simulink model "Inverter_32V_2A"  (R2025b)
settings: Solver=VariableStepAuto  StartTime=0.0  StopTime=0.3  FixedStep=SPWM_Ts  RelTol=1e-3
model workspace (MAT data in the model file):
  AC_LoadResistance = 9.23760430703
  AD_TimeConstant = 0.00025
  AD_a = [1 -0.881765205117]
  AD_b = [2.95586987209 -2.95586987209]
  CL_AAComp = 1.00249999972
  CL_Kaw = 20
  CL_Ki = 1.6
  CL_Kp = 0.005
  CL_N = 200
  CL_Ts = 0.0001
  CL_Vref = 32
  CL_faa = 1000
  CL_fp = 50
  CL_mff = 0.94
  CL_mmax = 1
  CommonModeBias = 0.15
  CommonModeKp = 0.02
  CommonModeShift = 1
  ControlStartTime = 0.06
  DampingCapuF = 4.7
  DampingResistance = 30
  DeadtimeComp = 0.08
  DeadtimeCurrentBand = 0.2
  DutyFeedforward = 0
  DutyMax = 0.75
  FilterDCR = 0.3
  KiCurrentLoop = 5
  KiVoltageLoop = 5
  KpCurrentLoop = 0.08
  KpVoltageLoop = 0.2
  LoadConnectTime = 0.18
  MainFilterCapuF = 4.7
  PR_Gain = 1.25
  PR_a10 = [1 -1.99838562653 0.999372033695]
  PR_a11 = [1 -1.99817857535 0.999372066214]
  PR_a13 = [1 -1.99770539603 0.999372140529]
  PR_a16 = [1 -1.99684804391 0.99937227518]
  PR_a17 = [1 -1.99652293757 0.99937232624]
  PR_a19 = [1 -1.9958137982 0.999372437614]
  PR_a2 = [1 -1.99933241937 0.999371884997]
  PR_a4 = [1 -1.99921404574 0.999371903588]
  PR_a5 = [1 -1.99912527012 0.99937191753]
  PR_a7 = [1 -1.9988885544 0.999371954708]
  PR_a8 = [1 -1.99874062131 0.999371977941]
  PR_b10 = [0.236875635534 -0.472442728614 0.23556709308]
  PR_b11 = [0.215389811794 -0.429471148895 0.214081337101]
  PR_b13 = [0.182331988259 -0.363355656682 0.181023668423]
  PR_b16 = [0.148235597863 -0.295163156474 0.146927558611]
  PR_b17 = [0.139542977111 -0.277778021366 0.138235044255]
  PR_b19 = [0.124900915012 -0.248494129248 0.123593214235]
  PR_b2 = [0.425928775502 -0.847596177142 0.42166740164]
  PR_b4 = [0.279572378961 -0.55553023994 0.275957860979]
  PR_b5 = [0.246657018631 -0.490084248228 0.243427229597]
  PR_b7 = [0.202908225742 -0.403457656245 0.200549430503]
  PR_b8 = [0.186290317354 -0.370698545076 0.184408227722]
  PrechargeBypassTime = 0.16
  PrechargeResistance = 47
  RegenerativeMode = 1
  ReturnCurrent = 2
  ReturnRampTime = 0.08
  ReturnTs = 1e-05
  SPWM_Ndead = 10
  SPWM_Tdead = 2e-06
  SPWM_Ts = 2e-07
  SPWM_Vgate = 10
  SPWM_f1 = 50
  SPWM_fs = 20000
  SPWM_m = 0.8
  VoltageRampRate = 100
  op_snapshot1 : opcond.OperatingPoint (value not decoded)
  testadd = 0
undefined symbols (not defined in the file): DiscIntNeverNeededParam, dspblkCoreblockFVToolHelper, gcbh
libraries: fl_lib x31, ee_lib x30, nesl_utility x26, simulink x1
(part 2 of 2)

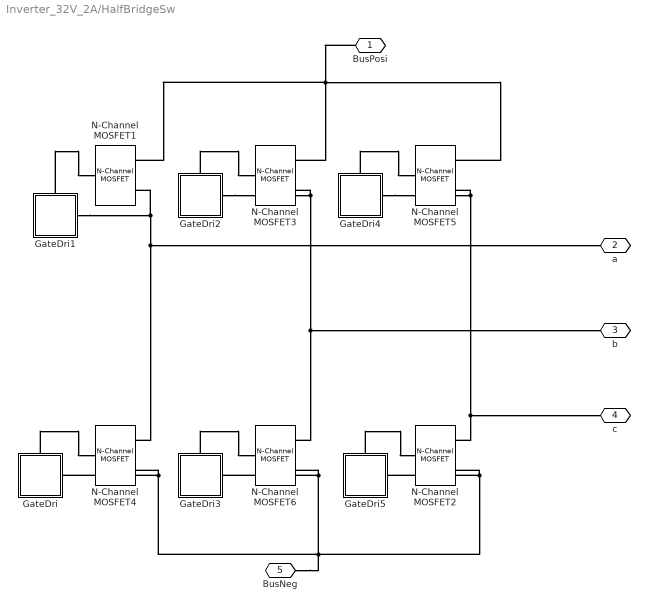
== system Inverter_32V_2A/HalfBridgeSw ==
  GateDri : Subsystem
      settings: PortSchema="{\"entries\":[{\"content\":{\"sides\":[{\"content\":{\"connectorIds\":[\"LConn1\"]},\"type\":\"ConnectorPlacement.EquallySpacedRectSide\",\"uuid\":\"5ec2b66a-2e5f-4a29-ad7d-11e5a28469f4\"},{\"content\":{\"side\":\"RIGHT\"},\"type\":\"ConnectorPlacement.EquallySpacedRectSide\",\"uuid\":\"968cf12b-ade8-46ac-9f94-1e8ea2f3f677\"},{\"content\":{\"side\":\"TOP\"},\"type\":\"ConnectorPlacement.EquallySpacedRectSide\",\"uuid\":\"41030f6a-5ac0-4230-aa4b-0c03378f97d6\"},{\"content\":{\"connectorIds\":[\"RConn1\"],\"side\":\"BOTTOM\"},\"type\":\"ConnectorPlacement.EquallySpacedRectSide\",\"uuid\":\"8f964c8e-6f21-4ad0-8f7c-edbb0b22c660\"}]},\"type\":\"ConnectorPlacement.EquallySpacedConnector\",\"uuid\":\"dccfb76b-3882-476d-8e51-da801e2932e6\"}],\"packageUris\":[\"http://schema.mathworks.com/mf0/Connector/R2020b\"],\"version\":\"1.0\"}"
  GateDri1 : Subsystem
      settings: PortSchema="{\"entries\":[{\"content\":{\"sides\":[{\"content\":{\"connectorIds\":[\"LConn1\"]},\"type\":\"ConnectorPlacement.EquallySpacedRectSide\",\"uuid\":\"5ec2b66a-2e5f-4a29-ad7d-11e5a28469f4\"},{\"content\":{\"side\":\"RIGHT\"},\"type\":\"ConnectorPlacement.EquallySpacedRectSide\",\"uuid\":\"968cf12b-ade8-46ac-9f94-1e8ea2f3f677\"},{\"content\":{\"side\":\"TOP\"},\"type\":\"ConnectorPlacement.EquallySpacedRectSide\",\"uuid\":\"41030f6a-5ac0-4230-aa4b-0c03378f97d6\"},{\"content\":{\"connectorIds\":[\"RConn1\"],\"side\":\"BOTTOM\"},\"type\":\"ConnectorPlacement.EquallySpacedRectSide\",\"uuid\":\"8f964c8e-6f21-4ad0-8f7c-edbb0b22c660\"}]},\"type\":\"ConnectorPlacement.EquallySpacedConnector\",\"uuid\":\"dccfb76b-3882-476d-8e51-da801e2932e6\"}],\"packageUris\":[\"http://schema.mathworks.com/mf0/Connector/R2020b\"],\"version\":\"1.0\"}"
  GateDri2 : Subsystem
      settings: PortSchema="{\"entries\":[{\"content\":{\"sides\":[{\"content\":{\"connectorIds\":[\"LConn1\"]},\"type\":\"ConnectorPlacement.EquallySpacedRectSide\",\"uuid\":\"5ec2b66a-2e5f-4a29-ad7d-11e5a28469f4\"},{\"content\":{\"side\":\"RIGHT\"},\"type\":\"ConnectorPlacement.EquallySpacedRectSide\",\"uuid\":\"968cf12b-ade8-46ac-9f94-1e8ea2f3f677\"},{\"content\":{\"side\":\"TOP\"},\"type\":\"ConnectorPlacement.EquallySpacedRectSide\",\"uuid\":\"41030f6a-5ac0-4230-aa4b-0c03378f97d6\"},{\"content\":{\"connectorIds\":[\"RConn1\"],\"side\":\"BOTTOM\"},\"type\":\"ConnectorPlacement.EquallySpacedRectSide\",\"uuid\":\"8f964c8e-6f21-4ad0-8f7c-edbb0b22c660\"}]},\"type\":\"ConnectorPlacement.EquallySpacedConnector\",\"uuid\":\"dccfb76b-3882-476d-8e51-da801e2932e6\"}],\"packageUris\":[\"http://schema.mathworks.com/mf0/Connector/R2020b\"],\"version\":\"1.0\"}"
  GateDri3 : Subsystem
      settings: PortSchema="{\"entries\":[{\"content\":{\"sides\":[{\"content\":{\"connectorIds\":[\"LConn1\"]},\"type\":\"ConnectorPlacement.EquallySpacedRectSide\",\"uuid\":\"5ec2b66a-2e5f-4a29-ad7d-11e5a28469f4\"},{\"content\":{\"side\":\"RIGHT\"},\"type\":\"ConnectorPlacement.EquallySpacedRectSide\",\"uuid\":\"968cf12b-ade8-46ac-9f94-1e8ea2f3f677\"},{\"content\":{\"side\":\"TOP\"},\"type\":\"ConnectorPlacement.EquallySpacedRectSide\",\"uuid\":\"41030f6a-5ac0-4230-aa4b-0c03378f97d6\"},{\"content\":{\"connectorIds\":[\"RConn1\"],\"side\":\"BOTTOM\"},\"type\":\"ConnectorPlacement.EquallySpacedRectSide\",\"uuid\":\"8f964c8e-6f21-4ad0-8f7c-edbb0b22c660\"}]},\"type\":\"ConnectorPlacement.EquallySpacedConnector\",\"uuid\":\"dccfb76b-3882-476d-8e51-da801e2932e6\"}],\"packageUris\":[\"http://schema.mathworks.com/mf0/Connector/R2020b\"],\"version\":\"1.0\"}"
  GateDri4 : Subsystem
      settings: PortSchema="{\"entries\":[{\"content\":{\"sides\":[{\"content\":{\"connectorIds\":[\"LConn1\"]},\"type\":\"ConnectorPlacement.EquallySpacedRectSide\",\"uuid\":\"5ec2b66a-2e5f-4a29-ad7d-11e5a28469f4\"},{\"content\":{\"side\":\"RIGHT\"},\"type\":\"ConnectorPlacement.EquallySpacedRectSide\",\"uuid\":\"968cf12b-ade8-46ac-9f94-1e8ea2f3f677\"},{\"content\":{\"side\":\"TOP\"},\"type\":\"ConnectorPlacement.EquallySpacedRectSide\",\"uuid\":\"41030f6a-5ac0-4230-aa4b-0c03378f97d6\"},{\"content\":{\"connectorIds\":[\"RConn1\"],\"side\":\"BOTTOM\"},\"type\":\"ConnectorPlacement.EquallySpacedRectSide\",\"uuid\":\"8f964c8e-6f21-4ad0-8f7c-edbb0b22c660\"}]},\"type\":\"ConnectorPlacement.EquallySpacedConnector\",\"uuid\":\"dccfb76b-3882-476d-8e51-da801e2932e6\"}],\"packageUris\":[\"http://schema.mathworks.com/mf0/Connector/R2020b\"],\"version\":\"1.0\"}"
  GateDri5 : Subsystem
      settings: PortSchema="{\"entries\":[{\"content\":{\"sides\":[{\"content\":{\"connectorIds\":[\"LConn1\"]},\"type\":\"ConnectorPlacement.EquallySpacedRectSide\",\"uuid\":\"5ec2b66a-2e5f-4a29-ad7d-11e5a28469f4\"},{\"content\":{\"side\":\"RIGHT\"},\"type\":\"ConnectorPlacement.EquallySpacedRectSide\",\"uuid\":\"968cf12b-ade8-46ac-9f94-1e8ea2f3f677\"},{\"content\":{\"side\":\"TOP\"},\"type\":\"ConnectorPlacement.EquallySpacedRectSide\",\"uuid\":\"41030f6a-5ac0-4230-aa4b-0c03378f97d6\"},{\"content\":{\"connectorIds\":[\"RConn1\"],\"side\":\"BOTTOM\"},\"type\":\"ConnectorPlacement.EquallySpacedRectSide\",\"uuid\":\"8f964c8e-6f21-4ad0-8f7c-edbb0b22c660\"}]},\"type\":\"ConnectorPlacement.EquallySpacedConnector\",\"uuid\":\"dccfb76b-3882-476d-8e51-da801e2932e6\"}],\"packageUris\":[\"http://schema.mathworks.com/mf0/Connector/R2020b\"],\"version\":\"1.0\"}"
  N-Channel MOSFET{1..6} (6 alike) : ee_lib/Semiconductors & Converters/N-Channel MOSFET  paramTerminal=ee.enum.mosfet.numberOfTerminals.three  parameterization=ee.enum.mosfet.parameterization.datasheet  Beta=5.0 A/V^2  Rds=0.025 Ohm  Id=6.0 A  Vgs=10 V  Vth=1.7 V  Vth0=1.7 V  lam=0 1/V  gamma_vth=0.5 V^(1/2)  phib=0.5 V  Vth1=1.9071 V  Vbs1=-1 V  Vth2=2.066 V  Vbs2=-2 V  Tmeas=25 degC  Vgs_vec=[-1, -.5, 2, 3, 4, 5] V  Vds_vec=[0, 2, 4, 8, 12, 16, 20] V  Vbs_vec=[0, -4, -6, -12] V  T_vec=[25, 125] degC  Vth_vec=[.4, 1.2, 1.4, 1.45] V  Vth_mat=[.4, .35; 1.2, 1.15; 1.4, 1.35; 1.45, 1.4] V  Ids_mat=[0, 0, 0, 0, 0, 0, 0; 0, 0, 0, 0, 0, 0, 0; 0, .003, .0038, .0043, .0046, .0048, .0049; 0, .0055, .008, .009, .0095, .01, .0101; 0, .0115, .016, .018, .019, .0195, .02; 0, .0152, .0225, .0265, .028, .0295, .03] A  Ids_mat0=[0, 0, 0, 0, 0, 0, 0; 0, 0, 0, 0, 0, 0, 0; 0, .003, .0038, .0043, .0046, .0048, .0049; 0, .0055, .008, .009, .0095, .01, .0101; 0, .0115, .016, .018, .019, .0195, .02; 0, .0152, .0225, .0265, .028, .0295, .03] A  Ids_mat_3D=zeros(6, 7, 2) A  Ids_mat_3D0=zeros(6, 7, 2) A  IV_table_symmetry=ee.enum.mosfet.symmetricNIV.no  RS=0.0001 Ohm  RD=0.01 Ohm  RB=0.001 Ohm  LeadRs=0 Ohm  LeadRd=0 Ohm  LeadRg=0 Ohm  LeadRb=0 Ohm  LS=0 nH  LD=0 nH  LG=0 nH  LB=0 nH  C_param=ee.enum.mosfet.capacitanceParam.fixedciss  C_GS=270 pF  C_GD=80 pF  C_GB=0 pF  C_DS=0 pF  C_iss=350 pF  C_rss=80 pF  C_oss=0 pF  C_iss_vec=[720, 700, 590, 470, 390, 310] pF  C_rss_vec=[450, 400, 300, 190, 95, 55] pF  C_oss_vec=[900, 810, 690, 420, 270, 170] pF  C_GS_vec=[270, 300, 290, 280, 295, 255] pF  C_GD_vec=[450, 400, 300, 190, 95, 55] pF  C_GB_vec=[270, 300, 290, 280, 295, 255] pF  C_Vgs_vec=0 V  C_DS_vec=[450, 410, 390, 230, 175, 115] pF  C_Vds_vec=[.1, .3, 1, 3, 10, 30] V  V_GS_for_cap_data=0 V  charge_linearity_param=ee.enum.mosfet.cgdLinearity.constant  C_OX=200 pF  V_C_OX=-0.5 V  charge_linearity_param_vgb=ee.enum.mosfet.cgbLinearity.instantly  charge_linearity_param_with_vgb=ee.enum.mosfet.cgbLinearityWithSeparateCgb.instantly  Di_param=ee.enum.mosfet.diodeParam.exponential  IsDiode=1e-12 A  Vbi=0.6 V  n=1  Cj0Diode=0 pF  TT=50e-9 s  Tmeas_dio=25 degC  TableTypeNoT=ee.enum.mosfet.tableType.IfMat  TableType=ee.enum.diode.tableType.IfMat  IfVec=[.07, .12, .19, 1.75, 4.24, 7.32, 11.2] A  IfMat=[.07, .12, .19, 1.75, 4.24, 7.32, 11.2; .16, .3, .72, 2.14, 4.02, 6.35, 9.12] A  VfVecV=[.9, 1.15, 1.25, 1.5, 1.75, 2.17, 2.6, 2.85] V  VfMatV=[.9, 1.15, 1.25, 1.5, 1.75, 2.17, 2.6, 2.85; .58, .68, .75, 1.1, 1.38, 1.77, 2.27, 2.7] V  TjVec=[25, 125] degC  VfVec=[.5, .7, .9, 1.3, 1.7, 2.1, 2.5] V  IfVecV=[.1, .2, .5, 1, 2, 4, 7, 10] A  diode_Goff=1e-12 1/Ohm  prmDatasheet=ee.enum.temperatureParameterization.simulation  prmEquCoeff=ee.enum.temperatureParameterization.none  dVth_dT=-6 mV/K  dVth0_dT=-6 mV/K  Rds_T2=0.037 Ohm  BEXDatasheet=-1.5  BEXEquCoeff=-1.5  etaisDatasheet=3  etaisEquCoeff=3  Tmeas2=125 degC  etaisTabulated=3  TdeviceDatasheet=25 degC  TdeviceEquCoeff=25 degC  TdeviceTabulated=25 degC  i_g_specify=off  i_g_priority=None  i_g=0 A  i_g_nominal_specify=off  i_g_nominal_value=1  i_g_nominal_unit=A  i_d_specify=off  i_d_priority=None  i_d=0 A  i_d_nominal_specify=off  i_d_nominal_value=1  i_d_nominal_unit=A  i_b_specify=off  i_b_priority=None  i_b=0 A  i_b_nominal_specify=off  i_b_nominal_value=1  i_b_nominal_unit=A  voltage_gs_specify=off  voltage_gs_priority=None  voltage_gs=0 V  voltage_gs_nominal_specify=off  voltage_gs_nominal_value=1  voltage_gs_nominal_unit=V  voltage_ds_specify=off  voltage_ds_priority=None  voltage_ds=0 V  voltage_ds_nominal_specify=off  voltage_ds_nominal_value=1  voltage_ds_nominal_unit=V  voltage_bs_specify=off  voltage_bs_priority=None  voltage_bs=0 V  voltage_bs_nominal_specify=off  voltage_bs_nominal_value=1  voltage_bs_nominal_unit=V  v_Cgs_specify=off  v_Cgs_priority=High  v_Cgs=0 V  v_Cgs_nominal_specify=off  v_Cgs_nominal_value=1  v_Cgs_nominal_unit=V  v_Cds_specify=off  v_Cds_priority=High  v_Cds=0 V  v_Cds_nominal_specify=off  v_Cds_nominal_value=1  v_Cds_nominal_unit=V  v_Cbs_specify=off  v_Cbs_priority=High  v_Cbs=0 V  v_Cbs_nominal_specify=off  v_Cbs_nominal_value=1  v_Cbs_nominal_unit=V  thermal_network_parameterization=ee.enum.thermalNetworkTopology.junctionCase  Rth=[0, 10] K/W  Rth_Cauer=[1, 3, 10] K/W  Rth_Foster=[.08, .14, .22, .16] K/W  thermal_mass_parameterization=ee.enum.thermalNetwork.timeconstant  thermal_mass=[0, 1] J/K  thermal_mass_Cauer=[.1, .3, 1] J/K  thermal_mass_Foster=[.001, .005, .05, .5] J/K  thermal_time_constant=[0, 10] s  thermal_time_constant_Cauer=[1, 3, 10] s  thermal_time_constant_Foster=[7e-05, .0007, .01, .08] s  thermal_mass_initial_temperatures=[25, 25] degC  thermal_mass_initial_temperatures_Cauer=[25, 25, 25] degC  Tvec_initial_Foster=[25, 25, 25, 25] degC  betaref=18 A/V^2  Vfbref=-1.1 V  gamma=3.5 V^(1/2)  phib2ref=1 V  thesatref=0.4 1/V  alpha=0  Vp=5e-2 V  thesrref=0 1/V  m=8  Tref=25 degC  Rsref=2e-3 Ohm  Rdref=0.17 Ohm  Rgref=8.4 Ohm  Rbref=2e-3 Ohm  Cox=1500 pF  Cgso=100 pF  Cgdo=14 pF  Isref=5.2e-13 A  Cj0=480 pF  Tprm=1  etabet=1.3  Stvfb=5e-4 V/K  Stphib=-8.5e-4 V/K  etasat=1.04  etasr=0.65  etar=0.95  etais=3  Tsim=25 degC  Ig_specify=off  Ig_priority=None  Ig=0 A  Ig_nominal_specify=off  Ig_nominal_value=1  Ig_nominal_unit=nA  Ids_specify=off  Ids_priority=None  Ids=0 A  Ids_nominal_specify=off  Ids_nominal_value=1  Ids_nominal_unit=A  Ib_specify=off  Ib_priority=None  Ib=0 A  Ib_nominal_specify=off  Ib_nominal_value=1  Ib_nominal_unit=uA  V_gs_specify=off  V_gs_priority=None  V_gs=0 V  V_gs_nominal_specify=off  V_gs_nominal_value=1  V_gs_nominal_unit=V  V_ds_specify=off  V_ds_priority=None  V_ds=0 V  V_ds_nominal_specify=off  V_ds_nominal_value=1  V_ds_nominal_unit=V  V_bs_specify=off  V_bs_priority=None  V_bs=0 V  V_bs_nominal_specify=off  V_bs_nominal_value=1  V_bs_nominal_unit=V  QGoverCox_specify=off  QGoverCox_priority=None  QGoverCox=0 V  QGoverCox_nominal_specify=off  QGoverCox_nominal_value=1  QGoverCox_nominal_unit=V  QDoverCox_specify=off  QDoverCox_priority=None  QDoverCox=0 V  QDoverCox_nominal_specify=off  QDoverCox_nominal_value=1  QDoverCox_nominal_unit=V  QBoverCox_specify=off  QBoverCox_priority=None  QBoverCox=0 V  QBoverCox_nominal_specify=off  QBoverCox_nominal_value=1  QBoverCox_nominal_unit=V  T0=[25, 25] degC  T0_Cauer=[25, 25, 25] degC
  BusPosi : PMIOPort  Side=Left
  a : PMIOPort  Port=2  Side=Right
  b : PMIOPort  Port=3  Side=Right
  c : PMIOPort  Port=4  Side=Right
  BusNeg : PMIOPort  Port=5  Side=Right
  connections:
  GateDri3/LConn1 -- N-Channel MOSFET6/LConn1
  GateDri4/RConn1 -- c/RConn1 -- N-Channel MOSFET2/RConn1 -- N-Channel MOSFET5/RConn2
  GateDri1/RConn1 -- N-Channel MOSFET1/RConn2 -- a/RConn1 -- N-Channel MOSFET4/RConn1
  GateDri5/RConn1 -- GateDri/RConn1 -- N-Channel MOSFET4/RConn2 -- N-Channel MOSFET6/RConn2 -- GateDri3/RConn1 -- BusNeg/RConn1 -- N-Channel MOSFET2/RConn2
  N-Channel MOSFET1/RConn1 -- N-Channel MOSFET5/RConn1 -- N-Channel MOSFET3/RConn1 -- BusPosi/RConn1
  GateDri/LConn1 -- N-Channel MOSFET4/LConn1
  GateDri4/LConn1 -- N-Channel MOSFET5/LConn1
  GateDri1/LConn1 -- N-Channel MOSFET1/LConn1
  N-Channel MOSFET3/RConn2 -- b/RConn1 -- N-Channel MOSFET6/RConn1 -- GateDri2/RConn1
  GateDri5/LConn1 -- N-Channel MOSFET2/LConn1
  GateDri2/LConn1 -- N-Channel MOSFET3/LConn1

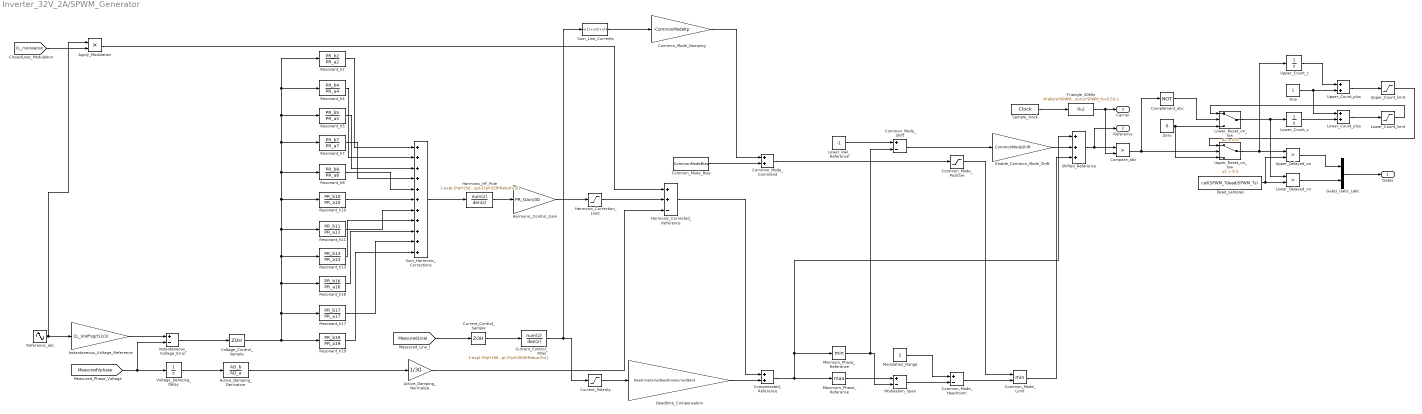
== system Inverter_32V_2A/SPWM_Generator ==
  Active_Damping_Derivative : DiscreteTransferFcn  Numerator=AD_b  Denominator=AD_a  SampleTime=ReturnTs
  Active_Damping_Normalize : Gain  Gain=1/30
  Apply_Modulation : Product
  Common_Mode_Bias : Constant  Value=CommonModeBias
  Common_Mode_Command : Sum
  Common_Mode_Damping : Gain  Gain=-CommonModeKp
  Common_Mode_Headroom : Sum  Inputs=+-
  Common_Mode_Limit : MinMax  Inputs=2
  Common_Mode_Positive : Saturate  UpperLimit=2  LowerLimit=0
  Common_Mode_Shift : Sum  Inputs=+-
  Compare_abc : RelationalOperator  Operator=>  OutDataTypeStr=boolean  RndMeth=Simplest  InputSameDT=off
  Compensated_Reference : Sum
  Complement_abc : Logic  Operator=NOT  Inputs=1  IconShape=distinctive  AllPortsSameDT=off  OutDataTypeStr=boolean
  Current_Control_Filter : DiscreteTransferFcn  Numerator=1-exp(-2*pi*2000*ReturnTs)  Denominator=[1 -exp(-2*pi*2000*ReturnTs)]  SampleTime=ReturnTs
  Current_Control_Sample : ZeroOrderHold  SampleTime=ReturnTs
  Current_Polarity : Saturate  UpperLimit=DeadtimeCurrentBand  LowerLimit=-DeadtimeCurrentBand
  Dead_samples : Constant  Value=ceil(SPWM_Tdead/SPWM_Ts)
  Deadtime_Compensation : Gain  Gain=DeadtimeComp/DeadtimeCurrentBand
  Enable_Common_Mode_Shift : Gain  Gain=CommonModeShift
  Gates_Uabc_Labc : Mux  Inputs=2
  Harmonic_Control_Gain : Gain  Gain=PR_Gain/30
  Harmonic_Corrected_Reference : Sum  Inputs=++-
  Harmonic_Correction_Limit : Saturate  UpperLimit=0.15  LowerLimit=-0.15
  Harmonic_HF_Pole : DiscreteTransferFcn  Numerator=1-exp(-2*pi*250*ReturnTs)  Denominator=[1 -exp(-2*pi*250*ReturnTs)]  SampleTime=ReturnTs
  Instantaneous_Voltage_Error : Sum  Inputs=+-
  Instantaneous_Voltage_Reference : Gain  Gain=CL_Vref*sqrt(2/3)
  Lower_Count_limit : Saturate  UpperLimit=ceil(SPWM_Tdead/SPWM_Ts)+1  LowerLimit=0
  Lower_Count_plus : Sum
  Lower_Count_z : UnitDelay  InitialCondition=[0 0 0]  SampleTime=SPWM_Ts  HasFrameUpgradeWarning=on
  Lower_Delayed_on : RelationalOperator  Operator=>  OutDataTypeStr=boolean  RndMeth=Simplest  InputSameDT=off
  Lower_Rail_Reference : Constant  Value=-1
  Lower_Reset_on_low : Switch  Criteria=u2 > Threshold  Threshold=0.5  SaturateOnIntegerOverflow=off  InputSameDT=off
  Maximum_Phase_Reference : MinMax  Function=max
  Minimum_Phase_Reference : MinMax
  Modulation_Range : Constant  Value=2
  Modulation_Span : Sum  Inputs=+-
  One : Constant
  Reference_abc : Sin  Frequency=2*pi*SPWM_f1  Phase=[0 -2*pi/3 2*pi/3]  SampleTime=SPWM_Ts
  Resonant_h10 : DiscreteTransferFcn  Numerator=PR_b10  Denominator=PR_a10  SampleTime=ReturnTs
  Resonant_h11 : DiscreteTransferFcn  Numerator=PR_b11  Denominator=PR_a11  SampleTime=ReturnTs
  Resonant_h13 : DiscreteTransferFcn  Numerator=PR_b13  Denominator=PR_a13  SampleTime=ReturnTs
  Resonant_h16 : DiscreteTransferFcn  Numerator=PR_b16  Denominator=PR_a16  SampleTime=ReturnTs
  Resonant_h17 : DiscreteTransferFcn  Numerator=PR_b17  Denominator=PR_a17  SampleTime=ReturnTs
  Resonant_h19 : DiscreteTransferFcn  Numerator=PR_b19  Denominator=PR_a19  SampleTime=ReturnTs
  Resonant_h2 : DiscreteTransferFcn  Numerator=PR_b2  Denominator=PR_a2  SampleTime=ReturnTs
  Resonant_h4 : DiscreteTransferFcn  Numerator=PR_b4  Denominator=PR_a4  SampleTime=ReturnTs
  Resonant_h5 : DiscreteTransferFcn  Numerator=PR_b5  Denominator=PR_a5  SampleTime=ReturnTs
  Resonant_h7 : DiscreteTransferFcn  LoadFcn=dspblkCoreblockFVToolHelper(gcbh,'load');  Numerator=PR_b7  Denominator=PR_a7  SampleTime=ReturnTs
      settings: CopyFcn=dspblkCoreblockFVToolHelper(gcbh,'copy');  DeleteFcn=dspblkCoreblockFVToolHelper(gcbh,'close');  ModelCloseFcn=dspblkCoreblockFVToolHelper(gcbh,'close');  PreSaveFcn=dspblkCoreblockFVToolHelper(gcbh,'presave');  PostSaveFcn=dspblkCoreblockFVToolHelper(gcbh,'postsave');  CloseFcn=dspblkCoreblockFVToolHelper(gcbh,'close');
  Resonant_h8 : DiscreteTransferFcn  LoadFcn=dspblkCoreblockFVToolHelper(gcbh,'load');  Numerator=PR_b8  Denominator=PR_a8  SampleTime=ReturnTs
      settings: CopyFcn=dspblkCoreblockFVToolHelper(gcbh,'copy');  DeleteFcn=dspblkCoreblockFVToolHelper(gcbh,'close');  ModelCloseFcn=dspblkCoreblockFVToolHelper(gcbh,'close');  PreSaveFcn=dspblkCoreblockFVToolHelper(gcbh,'presave');  PostSaveFcn=dspblkCoreblockFVToolHelper(gcbh,'postsave');  CloseFcn=dspblkCoreblockFVToolHelper(gcbh,'close');
  Sample_clock : DigitalClock  SampleTime=SPWM_Ts
  Shifted_Reference : Sum  Inputs=+++
  Sum_Harmonic_Corrections : Sum  Inputs=+++++++++++
  Sum_Line_Currents : Fcn  Expr=u(1)+u(2)+u(3)
  Triangle_20kHz : Fcn  Expr=4*abs(u*SPWM_fs-floor(u*SPWM_fs+0.5))-1
  Upper_Count_limit : Saturate  UpperLimit=ceil(SPWM_Tdead/SPWM_Ts)+1  LowerLimit=0
  Upper_Count_plus : Sum
  Upper_Count_z : UnitDelay  InitialCondition=[0 0 0]  SampleTime=SPWM_Ts  HasFrameUpgradeWarning=on
  Upper_Delayed_on : RelationalOperator  Operator=>  OutDataTypeStr=boolean  RndMeth=Simplest  InputSameDT=off
  Upper_Reset_on_low : Switch  Criteria=u2 > Threshold  Threshold=0.5  SaturateOnIntegerOverflow=off  InputSameDT=off
  Voltage_Control_Sample : ZeroOrderHold  SampleTime=ReturnTs
  Voltage_Damping_Delay : UnitDelay  SampleTime=ReturnTs  HasFrameUpgradeWarning=on
  Zero : Constant  Value=0
  Gates : Outport
  Reference : Outport  Port=2
  Carrier : Outport  Port=3
  wires:
  Current_Control_Filter/1 -> Current_Polarity/1, Sum_Line_Currents/1
  Apply_Modulation/1 -> Harmonic_Corrected_Reference/1
  Complement_abc/1 -> Lower_Reset_on_low/2
  [CL_modulation] -> Apply_Modulation/2
  Upper_Count_limit/1 -> Upper_Reset_on_low/1
  Current_Control_Sample/1 -> Current_Control_Filter/1
  Reference_abc/1 -> Apply_Modulation/1, Instantaneous_Voltage_Reference/1
  Zero/1 -> Upper_Reset_on_low/3, Lower_Reset_on_low/3
  Resonant_h10/1 -> Sum_Harmonic_Corrections/6
  Instantaneous_Voltage_Reference/1 -> Instantaneous_Voltage_Error/1
  [MeasuredVphase] -> Voltage_Damping_Delay/1, Instantaneous_Voltage_Error/2
  Instantaneous_Voltage_Error/1 -> Voltage_Control_Sample/1
  Voltage_Control_Sample/1 -> Resonant_h4/1, Resonant_h2/1, Resonant_h5/1, Resonant_h7/1, Resonant_h8/1, Resonant_h10/1, Resonant_h11/1, Resonant_h13/1, Resonant_h16/1, Resonant_h17/1, Resonant_h19/1
  Voltage_Damping_Delay/1 -> Active_Damping_Derivative/1
  Active_Damping_Derivative/1 -> Active_Damping_Normalize/1
  [MeasuredLineI] -> Current_Control_Sample/1
  Resonant_h2/1 -> Sum_Harmonic_Corrections/1
  Harmonic_Corrected_Reference/1 -> Compensated_Reference/1
  Sample_clock/1 -> Triangle_20kHz/1
  Resonant_h4/1 -> Sum_Harmonic_Corrections/2
  Upper_Count_plus/1 -> Upper_Count_limit/1
  Lower_Reset_on_low/1 -> Lower_Count_z/1, Lower_Delayed_on/1
  Resonant_h5/1 -> Sum_Harmonic_Corrections/3
  Gates_Uabc_Labc/1 -> Gates/1
  Resonant_h7/1 -> Sum_Harmonic_Corrections/4
  Resonant_h17/1 -> Sum_Harmonic_Corrections/10
  Resonant_h8/1 -> Sum_Harmonic_Corrections/5
  Resonant_h11/1 -> Sum_Harmonic_Corrections/7
  Resonant_h13/1 -> Sum_Harmonic_Corrections/8
  Lower_Count_plus/1 -> Lower_Count_limit/1
  Compare_abc/1 -> Upper_Reset_on_low/2, Complement_abc/1
  Resonant_h16/1 -> Sum_Harmonic_Corrections/9
  Lower_Rail_Reference/1 -> Common_Mode_Shift/1
  Harmonic_HF_Pole/1 -> Harmonic_Control_Gain/1
  Resonant_h19/1 -> Sum_Harmonic_Corrections/11
  Sum_Harmonic_Corrections/1 -> Harmonic_HF_Pole/1
  Enable_Common_Mode_Shift/1 -> Shifted_Reference/2
  Common_Mode_Positive/1 -> Common_Mode_Limit/1
  Active_Damping_Normalize/1 -> Harmonic_Corrected_Reference/3
  Harmonic_Control_Gain/1 -> Harmonic_Correction_Limit/1
  Sum_Line_Currents/1 -> Common_Mode_Damping/1
  Harmonic_Correction_Limit/1 -> Harmonic_Corrected_Reference/2
  Upper_Reset_on_low/1 -> Upper_Count_z/1, Upper_Delayed_on/1
  Current_Polarity/1 -> Deadtime_Compensation/1
  Dead_samples/1 -> Upper_Delayed_on/2, Lower_Delayed_on/2
  Common_Mode_Damping/1 -> Common_Mode_Command/1
  Common_Mode_Bias/1 -> Common_Mode_Command/2
  Deadtime_Compensation/1 -> Compensated_Reference/2
  Common_Mode_Command/1 -> Common_Mode_Positive/1
  Compensated_Reference/1 -> Shifted_Reference/1, Minimum_Phase_Reference/1, Maximum_Phase_Reference/1
  Minimum_Phase_Reference/1 -> Common_Mode_Shift/2, Modulation_Span/2
  Maximum_Phase_Reference/1 -> Modulation_Span/1
  Common_Mode_Headroom/1 -> Common_Mode_Limit/2
  Common_Mode_Shift/1 -> Enable_Common_Mode_Shift/1
  Common_Mode_Limit/1 -> Shifted_Reference/3
  Modulation_Range/1 -> Common_Mode_Headroom/1
  Modulation_Span/1 -> Common_Mode_Headroom/2
  Triangle_20kHz/1 -> Compare_abc/2, Carrier/1
  Shifted_Reference/1 -> Compare_abc/1, Reference/1
  Lower_Delayed_on/1 -> Gates_Uabc_Labc/2
  Upper_Count_z/1 -> Upper_Count_plus/1
  One/1 -> Upper_Count_plus/2, Lower_Count_plus/1
  Lower_Count_z/1 -> Lower_Count_plus/2
  Upper_Delayed_on/1 -> Gates_Uabc_Labc/1
  Lower_Count_limit/1 -> Lower_Reset_on_low/1

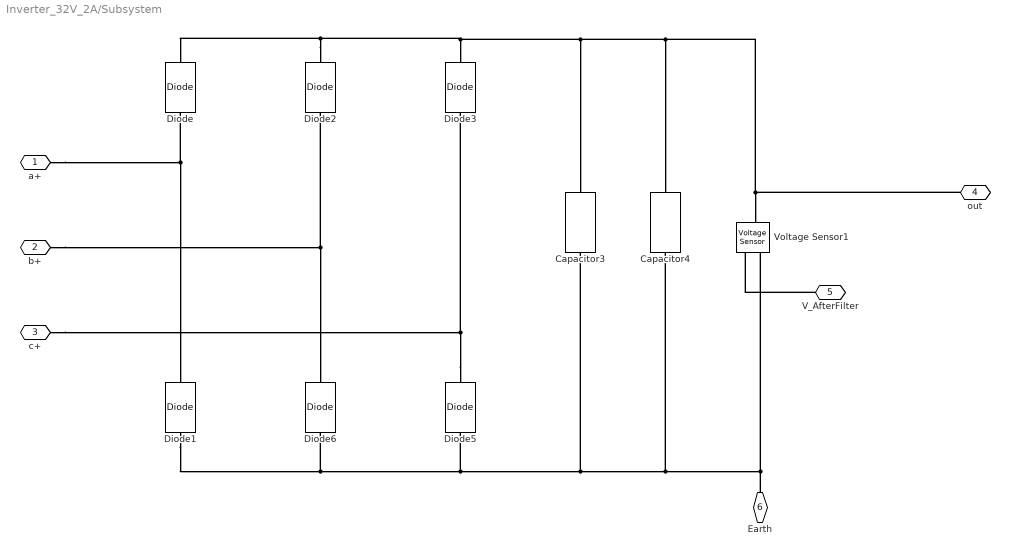
== system Inverter_32V_2A/Subsystem ==
  Capacitor3 : ee_lib/Passive/Capacitor  cap_option=ee.enum.passive.capacitor.capOption.const  c=1 uF  Cvec=[1e-05, 1e-06] F  Vvec=[0, 10] V  CV_table_symmetry=ee.enum.passive.capacitor.tableSymmetry.yes  f_vec=[1, 10] kHz  DFext_vec=[.8, 1.2]  enable_C_tol=ee.enum.toleranceApplication.none  averaging_period=0 s  C_tol=5  tol_distribution=ee.enum.toleranceDistribution.uniform  nSigma=4  r=0.1 Ohm  g=0 1/Ohm  enable_operating_limits=ee.enum.enable.no  operating_limit_action=ee.enum.passive.reportOpLim.warn  max_working_voltage_range=[-25, 25] V  power_rating=1 W  maxTemperature=85 degC  thermalEnable=false  thermalMass=1 J/K  i_specify=off  i_priority=None  i=0 A  i_nominal_specify=off  i_nominal_value=1  i_nominal_unit=A  v_specify=off  v_priority=None  v=0 V  v_nominal_specify=off  v_nominal_value=1  v_nominal_unit=V  vc_specify=off  vc_priority=High  vc=0 V  vc_nominal_specify=off  vc_nominal_value=1  vc_nominal_unit=V  T_specify=off  T_priority=None  T=298.15 K  T_nominal_specify=off  T_nominal_value=1  T_nominal_unit=K
  Capacitor4 : ee_lib/Passive/Capacitor  cap_option=ee.enum.passive.capacitor.capOption.const  c=10 uF  Cvec=[1e-05, 1e-06] F  Vvec=[0, 10] V  CV_table_symmetry=ee.enum.passive.capacitor.tableSymmetry.yes  f_vec=[1, 10] kHz  DFext_vec=[.8, 1.2]  enable_C_tol=ee.enum.toleranceApplication.none  averaging_period=0 s  C_tol=5  tol_distribution=ee.enum.toleranceDistribution.uniform  nSigma=4  r=0.1 Ohm  g=0 1/Ohm  enable_operating_limits=ee.enum.enable.no  operating_limit_action=ee.enum.passive.reportOpLim.warn  max_working_voltage_range=[-25, 25] V  power_rating=1 W  maxTemperature=85 degC  thermalEnable=false  thermalMass=1 J/K  i_specify=off  i_priority=None  i=0 A  i_nominal_specify=off  i_nominal_value=1  i_nominal_unit=A  v_specify=off  v_priority=None  v=0 V  v_nominal_specify=off  v_nominal_value=1  v_nominal_unit=V  vc_specify=off  vc_priority=High  vc=0 V  vc_nominal_specify=off  vc_nominal_value=1  vc_nominal_unit=V  T_specify=off  T_priority=None  T=298.15 K  T_nominal_specify=off  T_nominal_value=1  T_nominal_unit=K
  Diode{,1..3,5..6} (6 alike) : ee_lib/Semiconductors & Converters/Diode  ModelType=ee.enum.diode.modelType.pwl  TableType=ee.enum.diode.tableType.IfMat  IfMat=[.07, .12, .19, 1.75, 4.24, 7.32, 11.2; .16, .3, .72, 2.14, 5.02, 8.35, 13.12] A  VfMat=[.9, 1.15, 1.25, 1.5, 1.75, 2.17, 2.6, 2.85; .58, .68, .75, 1.1, 1.38, 1.77, 2.27, 2.7] V  TjVec=[25, 125] degC  VfVec=[.5, .7, .9, 1.3, 1.7, 2.1, 2.5] V  IfVec=[.1, .2, .5, 1, 2, 4, 7, 10] A  IrMat=[1e-06, 2e-06, 5e-06, 1e-05, 2.5e-05, 5e-05, .0001; 2e-06, 5e-06, 1e-05, 4e-05, 8e-05, .0002, .0005] A  VrMat=[10, 100, 200, 250, 300, 325, 350; 10, 70, 160, 220, 270, 300, 320] V  VrVec=[10, 20, 40, 50, 70, 80, 100] V  IrVec=[1e-06, 2e-06, 5e-06, 1e-05, 2e-05, 5e-05, .0001] A  Vf=0.6 V  Ron=0.3 Ohm  Goff=1e-8 S  prmExp=ee.enum.diode.expParam.useTwo  I12=[.0137, .545] A  V12=[.6, .7] V  RS=0 Ohm  Tmeas=298.15 K  IS=1e-12 A  ec=1  I1=0.0137 A  V1=0.6 V  N_series=1  N_parallel=1  ZenerEnable=false  Rz=0.3 Ohm  BV=inf V  C_param=ee.enum.diode.capParam.fixed  CJ=0 pF  CJ0=5 pF  Vvec=[.1, 10, 100] V  Cvec=[3.5, 1, .4] pF  VJ=1 V  Mgrad=0.5  FC=0.5  Q_param=ee.enum.diode.recoveryParam.off  iRM=-7.15 A  iF=4 A  didt=-750 A/us  trr_factor=3  trr=115 ns  Qrr=150 nA*s  Vr=-600 V  Ls=150 nH  Erec=0.03 J  TT=50 ns  tau=100 ns  T_param=ee.enum.diode.temperatureParam.off  Tdevice=298.15 K  I1_T2=0.245 A  V1_T2=0.5 V  IS_T2=1.25e-7 A  Tmeas2=125 degC  XTI_param=ee.enum.diode.xtiParam.pn  XTI=3  EG_param=ee.enum.diode.egapParam.material_si  EG=1.11 eV  dBVdT=0 V/K  enable_fault_input=simscape.enum.onoff.off  i_specify=off  i_priority=None  i=0 A  i_nominal_specify=off  i_nominal_value=1  i_nominal_unit=A  v_specify=off  v_priority=None  v=0 V  v_nominal_specify=off  v_nominal_value=1  v_nominal_unit=V  v_capacitor_specify=off  v_capacitor_priority=None  v_capacitor=0 V  v_capacitor_nominal_specify=off  v_capacitor_nominal_value=1  v_capacitor_nominal_unit=V  Qj_specify=off  Qj_priority=High  Qj=0 C  Qj_nominal_specify=off  Qj_nominal_value=1  Qj_nominal_unit=C  i_diode_specify=off  i_diode_priority=None  i_diode=0 A  i_diode_nominal_specify=off  i_diode_nominal_value=1  i_diode_nominal_unit=A  v_diode_specify=off  v_diode_priority=None  v_diode=0 V  v_diode_nominal_specify=off  v_diode_nominal_value=1  v_diode_nominal_unit=V  i_capacitor_specify=off  i_capacitor_priority=None  i_capacitor=0 A  i_capacitor_nominal_specify=off  i_capacitor_nominal_value=1  i_capacitor_nominal_unit=A  power_dissipated_specify=off  power_dissipated_priority=None  power_dissipated=0 W  power_dissipated_nominal_specify=off  power_dissipated_nominal_value=1  power_dissipated_nominal_unit=W  fidelity_level=ee.enum.diode.fidelity.includeChargeDyn  rec_loss_model=ee.enum.diode.reverseRecoveryModel.fixed  ErecVal=0 J  scaleWithIandV=true  ErecMat=zeros(2, 3) J  TjrecVec=[298.15, 398.15] K  IfrecVec=[.1, 1, 10] A  IrecVal=10 A  VrecVal=10 V  tFilter=1 / 1000 / 100 s  thermal_network_parameterization=ee.enum.thermalNetworkTopology.junctionCase  Rth=[0, 10] K/W  Rth_Cauer=[1, 3, 10] K/W  Rth_Foster=[.08, .14, .22, .16] K/W  thermal_mass_parameterization=ee.enum.thermalNetwork.timeconstant  thermal_mass=[0, 1] J/K  thermal_mass_Cauer=[.1, .3, 1] J/K  thermal_mass_Foster=[.001, .005, .05, .5] J/K  thermal_time_constant=[0, 10] s  thermal_time_constant_Cauer=[1, 3, 10] s  thermal_time_constant_Foster=[7e-05, .0007, .01, .08] s  thermal_mass_initial_temperatures=[25, 25] degC  thermal_mass_initial_temperatures_Cauer=[25, 25, 25] degC  junction_thermal_mass=0.01 J/K  Tvec_initial_Foster=[25, 25, 25, 25] degC  no_thermal_network=0  junction_temperature_specify=off  junction_temperature_priority=None  junction_temperature=25 degC  junction_temperature_nominal_specify=off  junction_temperature_nominal_value=1  junction_temperature_nominal_unit=degC
  Voltage Sensor1 : fl_lib/Electrical/Electrical Sensors/Voltage Sensor
  a+ : PMIOPort  Side=Left
  b+ : PMIOPort  Port=2  Side=Left
  c+ : PMIOPort  Port=3  Side=Left
  out : PMIOPort  Port=4  Side=Right
  V_AfterFilter : PMIOPort  Port=5  Side=Right
  Earth : PMIOPort  Port=6  Side=Right
  connections:
  Diode5/RConn1 -- c+/RConn1 -- Diode3/LConn1
  Diode2/RConn1 -- out/RConn1 -- Voltage Sensor1/LConn1 -- Capacitor4/LConn1 -- Capacitor3/LConn1 -- Diode3/RConn1 -- Diode/RConn1
  Diode2/LConn1 -- b+/RConn1 -- Diode6/RConn1
  Diode/LConn1 -- a+/RConn1 -- Diode1/RConn1
  V_AfterFilter/RConn1 -- Voltage Sensor1/RConn1
  Diode6/LConn1 -- Capacitor3/RConn1 -- Capacitor4/RConn1 -- Voltage Sensor1/RConn2 -- Earth/RConn1 -- Diode5/LConn1 -- Diode1/LConn1

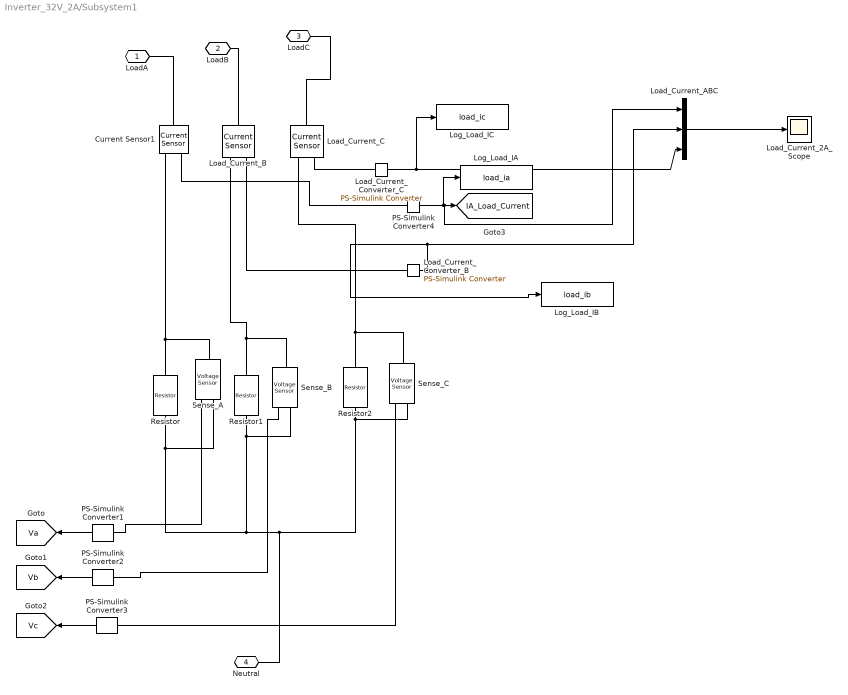
== system Inverter_32V_2A/Subsystem1 ==
  Current Sensor1 : fl_lib/Electrical/Electrical Sensors/Current Sensor
  Load_Current_2A_Scope : Scope
      settings: TimeSpan=0.45  ActiveDisplayYMinimum=0.46638614020950264  ActiveDisplayYMaximum=3.2365238393260536
  Load_Current_ABC : Mux  Inputs=3
  Load_Current_B : fl_lib/Electrical/Electrical Sensors/Current Sensor
  Load_Current_C : fl_lib/Electrical/Electrical Sensors/Current Sensor
  Load_Current_Converter_B : nesl_utility/PS-Simulink Converter  PhysicalDomain=network_engine_domain  SubClassName=ps_output  LeftPortType=input  RightPortType=output  PseudoPeriodic=off  Frequencies=[]  VectorFormat=inherit  Unit=inherit  AffineConversion=off
  Load_Current_Converter_C : nesl_utility/PS-Simulink Converter  PhysicalDomain=network_engine_domain  SubClassName=ps_output  LeftPortType=input  RightPortType=output  PseudoPeriodic=off  Frequencies=[]  VectorFormat=inherit  Unit=inherit  AffineConversion=off
  Log_Load_IA : ToWorkspace  VariableName=load_ia  SaveFormat=Timeseries  SampleTime=1e-5
  Log_Load_IB : ToWorkspace  VariableName=load_ib  SaveFormat=Timeseries  SampleTime=1e-5
  Log_Load_IC : ToWorkspace  VariableName=load_ic  SaveFormat=Timeseries  SampleTime=1e-5
  PS-Simulink Converter{1..4} (4 alike) : nesl_utility/PS-Simulink Converter  PhysicalDomain=network_engine_domain  SubClassName=ps_output  LeftPortType=input  RightPortType=output  PseudoPeriodic=off  Frequencies=[]  VectorFormat=inherit  Unit=inherit  AffineConversion=off
  Resistor : fl_lib/Electrical/Electrical Elements/Resistor  R=AC_LoadResistance*(1-RegenerativeMode)+1e9*RegenerativeMode Ohm  i_specify=off  i_priority=None  i=0 A  i_nominal_specify=off  i_nominal_value=1  i_nominal_unit=A  v_specify=off  v_priority=None  v=0 V  v_nominal_specify=off  v_nominal_value=1  v_nominal_unit=V
  Resistor1 : fl_lib/Electrical/Electrical Elements/Resistor  R=AC_LoadResistance*(1-RegenerativeMode)+1e9*RegenerativeMode Ohm  i_specify=off  i_priority=None  i=0 A  i_nominal_specify=off  i_nominal_value=1  i_nominal_unit=A  v_specify=off  v_priority=None  v=0 V  v_nominal_specify=off  v_nominal_value=1  v_nominal_unit=V
  Resistor2 : fl_lib/Electrical/Electrical Elements/Resistor  R=AC_LoadResistance*(1-RegenerativeMode)+1e9*RegenerativeMode Ohm  i_specify=off  i_priority=None  i=0 A  i_nominal_specify=off  i_nominal_value=1  i_nominal_unit=A  v_specify=off  v_priority=None  v=0 V  v_nominal_specify=off  v_nominal_value=1  v_nominal_unit=V
  Sense_A : fl_lib/Electrical/Electrical Sensors/Voltage Sensor
  Sense_B : fl_lib/Electrical/Electrical Sensors/Voltage Sensor
  Sense_C : fl_lib/Electrical/Electrical Sensors/Voltage Sensor
  LoadA : PMIOPort  Side=Left
  LoadB : PMIOPort  Port=2  Side=Left
  LoadC : PMIOPort  Port=3  Side=Left
  Neutral : PMIOPort  Port=4  Side=Right
  tag scope: IA_Load_Current=global, Va=global, Vb=global, Vc=global
  wires:
  PS-Simulink Converter3/1 -> [Vc]
  PS-Simulink Converter2/1 -> [Vb]
  PS-Simulink Converter1/1 -> [Va]
  Load_Current_ABC/1 -> Load_Current_2A_Scope/1
  PS-Simulink Converter4/1 -> Load_Current_ABC/1, [IA_Load_Current], Log_Load_IA/1
  Load_Current_Converter_B/1 -> Load_Current_ABC/2, Log_Load_IB/1
  Load_Current_Converter_C/1 -> Load_Current_ABC/3, Log_Load_IC/1
  connections:
  PS-Simulink Converter2/LConn1 -- Sense_B/RConn1
  PS-Simulink Converter1/LConn1 -- Sense_A/RConn1
  Current Sensor1/RConn2 -- Resistor/LConn1 -- Sense_A/LConn1
  PS-Simulink Converter3/LConn1 -- Sense_C/RConn1
  LoadA/RConn1 -- Current Sensor1/LConn1
  Load_Current_C/RConn2 -- Sense_C/LConn1 -- Resistor2/LConn1
  Load_Current_C/LConn1 -- LoadC/RConn1
  Load_Current_B/RConn2 -- Sense_B/LConn1 -- Resistor1/LConn1
  Load_Current_B/LConn1 -- LoadB/RConn1
  Neutral/RConn1 -- Resistor1/RConn1 -- Sense_B/RConn2 -- Resistor/RConn1 -- Sense_A/RConn2 -- Resistor2/RConn1 -- Sense_C/RConn2
  Load_Current_B/RConn1 -- Load_Current_Converter_B/LConn1
  Load_Current_C/RConn1 -- Load_Current_Converter_C/LConn1
  Current Sensor1/RConn1 -- PS-Simulink Converter4/LConn1

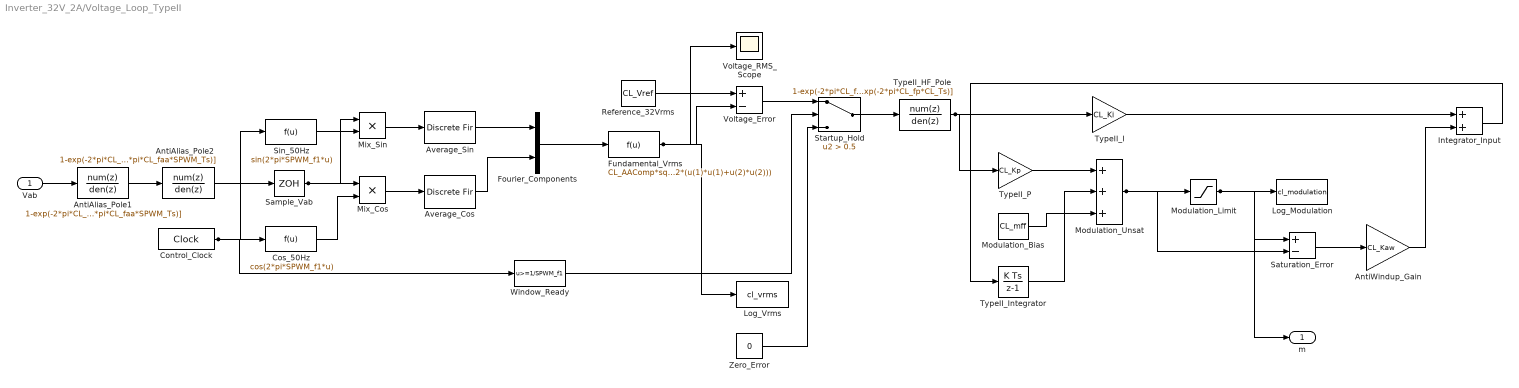
== system Inverter_32V_2A/Voltage_Loop_TypeII ==
  Vab : Inport
  AntiAlias_Pole1 : DiscreteTransferFcn  LoadFcn=dspblkCoreblockFVToolHelper(gcbh,'load');  Numerator=1-exp(-2*pi*CL_faa*SPWM_Ts)  Denominator=[1 -exp(-2*pi*CL_faa*SPWM_Ts)]  SampleTime=SPWM_Ts
      settings: CopyFcn=dspblkCoreblockFVToolHelper(gcbh,'copy');  DeleteFcn=dspblkCoreblockFVToolHelper(gcbh,'close');  ModelCloseFcn=dspblkCoreblockFVToolHelper(gcbh,'close');  PreSaveFcn=dspblkCoreblockFVToolHelper(gcbh,'presave');  PostSaveFcn=dspblkCoreblockFVToolHelper(gcbh,'postsave');  CloseFcn=dspblkCoreblockFVToolHelper(gcbh,'close');
  AntiAlias_Pole2 : DiscreteTransferFcn  LoadFcn=dspblkCoreblockFVToolHelper(gcbh,'load');  Numerator=1-exp(-2*pi*CL_faa*SPWM_Ts)  Denominator=[1 -exp(-2*pi*CL_faa*SPWM_Ts)]  SampleTime=SPWM_Ts
      settings: CopyFcn=dspblkCoreblockFVToolHelper(gcbh,'copy');  DeleteFcn=dspblkCoreblockFVToolHelper(gcbh,'close');  ModelCloseFcn=dspblkCoreblockFVToolHelper(gcbh,'close');  PreSaveFcn=dspblkCoreblockFVToolHelper(gcbh,'presave');  PostSaveFcn=dspblkCoreblockFVToolHelper(gcbh,'postsave');  CloseFcn=dspblkCoreblockFVToolHelper(gcbh,'close');
  AntiWindup_Gain : Gain  Gain=CL_Kaw
  Average_Cos : DiscreteFir  LoadFcn=dspblkCoreblockFVToolHelper(gcbh,'load');  Coefficients=ones(1,CL_N)/CL_N  SampleTime=CL_Ts
      settings: CopyFcn=dspblkCoreblockFVToolHelper(gcbh,'copy');  DeleteFcn=dspblkCoreblockFVToolHelper(gcbh,'close');  ModelCloseFcn=dspblkCoreblockFVToolHelper(gcbh,'close');  PreSaveFcn=dspblkCoreblockFVToolHelper(gcbh,'presave');  PostSaveFcn=dspblkCoreblockFVToolHelper(gcbh,'postsave');  CloseFcn=dspblkCoreblockFVToolHelper(gcbh,'close');
  Average_Sin : DiscreteFir  Coefficients=ones(1,CL_N)/CL_N  SampleTime=CL_Ts
  Control_Clock : DigitalClock  SampleTime=CL_Ts
  Cos_50Hz : Fcn  Expr=cos(2*pi*SPWM_f1*u)
  Fourier_Components : Mux  Inputs=2
  Fundamental_Vrms : Fcn  Expr=CL_AAComp*sqrt(2*(u(1)*u(1)+u(2)*u(2)))
  Integrator_Input : Sum
  Log_Modulation : ToWorkspace  VariableName=cl_modulation  SaveFormat=Timeseries  SampleTime=CL_Ts
  Log_Vrms : ToWorkspace  VariableName=cl_vrms  SaveFormat=Timeseries  SampleTime=CL_Ts
  Mix_Cos : Product
  Mix_Sin : Product
  Modulation_Bias : Constant  Value=CL_mff
  Modulation_Limit : Saturate  UpperLimit=CL_mmax  LowerLimit=0
  Modulation_Unsat : Sum  Inputs=+++
  Reference_32Vrms : Constant  Value=CL_Vref
  Sample_Vab : ZeroOrderHold  SampleTime=CL_Ts
  Saturation_Error : Sum  Inputs=+-
  Sin_50Hz : Fcn  Expr=sin(2*pi*SPWM_f1*u)
  Startup_Hold : Switch  Criteria=u2 > Threshold  Threshold=0.5  SaturateOnIntegerOverflow=off  InputSameDT=off
  TypeII_HF_Pole : DiscreteTransferFcn  LoadFcn=dspblkCoreblockFVToolHelper(gcbh,'load');  Numerator=1-exp(-2*pi*CL_fp*CL_Ts)  Denominator=[1 -exp(-2*pi*CL_fp*CL_Ts)]  SampleTime=CL_Ts
      settings: CopyFcn=dspblkCoreblockFVToolHelper(gcbh,'copy');  DeleteFcn=dspblkCoreblockFVToolHelper(gcbh,'close');  ModelCloseFcn=dspblkCoreblockFVToolHelper(gcbh,'close');  PreSaveFcn=dspblkCoreblockFVToolHelper(gcbh,'presave');  PostSaveFcn=dspblkCoreblockFVToolHelper(gcbh,'postsave');  CloseFcn=dspblkCoreblockFVToolHelper(gcbh,'close');
  TypeII_I : Gain  Gain=CL_Ki
  TypeII_Integrator : DiscreteIntegrator  SampleTime=CL_Ts  ICPrevOutput=DiscIntNeverNeededParam  ICPrevScaledInput=DiscIntNeverNeededParam
  TypeII_P : Gain  Gain=CL_Kp
  Voltage_Error : Sum  Inputs=+-
  Voltage_RMS_Scope : Scope
      settings: TimeSpan=0.45  ActiveDisplayYMinimum=0  ActiveDisplayYMaximum=36
  Window_Ready : Fcn  Expr=u>=1/SPWM_f1
  Zero_Error : Constant  Value=0
  m : Outport
  wires:
  AntiAlias_Pole2/1 -> Sample_Vab/1
  AntiAlias_Pole1/1 -> AntiAlias_Pole2/1
  Vab/1 -> AntiAlias_Pole1/1
  Fundamental_Vrms/1 -> Log_Vrms/1, Voltage_Error/2, Voltage_RMS_Scope/1
  Mix_Sin/1 -> Average_Sin/1
  Cos_50Hz/1 -> Mix_Cos/2
  Control_Clock/1 -> Window_Ready/1, Sin_50Hz/1, Cos_50Hz/1
  Sample_Vab/1 -> Mix_Sin/1, Mix_Cos/1
  TypeII_HF_Pole/1 -> TypeII_P/1, TypeII_I/1
  Sin_50Hz/1 -> Mix_Sin/2
  Integrator_Input/1 -> TypeII_Integrator/1
  Average_Sin/1 -> Fourier_Components/1
  Mix_Cos/1 -> Average_Cos/1
  Average_Cos/1 -> Fourier_Components/2
  Fourier_Components/1 -> Fundamental_Vrms/1
  Window_Ready/1 -> Startup_Hold/2
  Reference_32Vrms/1 -> Voltage_Error/1
  Voltage_Error/1 -> Startup_Hold/1
  Zero_Error/1 -> Startup_Hold/3
  Saturation_Error/1 -> AntiWindup_Gain/1
  Startup_Hold/1 -> TypeII_HF_Pole/1
  TypeII_P/1 -> Modulation_Unsat/1
  Modulation_Bias/1 -> Modulation_Unsat/3
  TypeII_Integrator/1 -> Modulation_Unsat/2
  Modulation_Unsat/1 -> Saturation_Error/2, Modulation_Limit/1
  TypeII_I/1 -> Integrator_Input/1
  Modulation_Limit/1 -> m/1, Log_Modulation/1, Saturation_Error/1
  AntiWindup_Gain/1 -> Integrator_Input/2

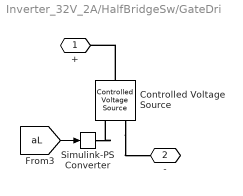
== system Inverter_32V_2A/HalfBridgeSw/GateDri ==
  Controlled Voltage Source : fl_lib/Electrical/Electrical Sources/Controlled Voltage Source
  Simulink-PS Converter : nesl_utility/Simulink-PS Converter  PhysicalDomain=network_engine_domain  SubClassName=ps_input  LeftPortType=input  RightPortType=output  PseudoPeriodic=off  Frequencies=[]  NoiseDistribution=none  NoiseParameters=[]  Unit=1  AffineConversion=off  FilteringAndDerivatives=provide  SimscapeFilterOrder=1  InputFilterTimeConstant=0.001  UdotUserProvided=0
  + : PMIOPort  Side=Left
  - : PMIOPort  Port=2  Side=Right
  wires:
  [aL] -> Simulink-PS Converter/1
  connections:
  Controlled Voltage Source/LConn1 -- +/RConn1
  Simulink-PS Converter/RConn1 -- Controlled Voltage Source/RConn1
  Controlled Voltage Source/RConn2 -- -/RConn1

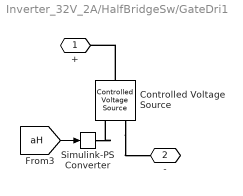
== system Inverter_32V_2A/HalfBridgeSw/GateDri1 ==
  Controlled Voltage Source : fl_lib/Electrical/Electrical Sources/Controlled Voltage Source
  Simulink-PS Converter : nesl_utility/Simulink-PS Converter  PhysicalDomain=network_engine_domain  SubClassName=ps_input  LeftPortType=input  RightPortType=output  PseudoPeriodic=off  Frequencies=[]  NoiseDistribution=none  NoiseParameters=[]  Unit=1  AffineConversion=off  FilteringAndDerivatives=provide  SimscapeFilterOrder=1  InputFilterTimeConstant=0.001  UdotUserProvided=0
  + : PMIOPort  Side=Left
  - : PMIOPort  Port=2  Side=Right
  wires:
  [aH] -> Simulink-PS Converter/1
  connections:
  Controlled Voltage Source/RConn2 -- -/RConn1
  Simulink-PS Converter/RConn1 -- Controlled Voltage Source/RConn1
  Controlled Voltage Source/LConn1 -- +/RConn1

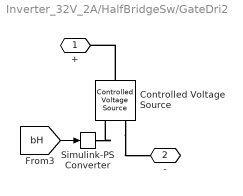
== system Inverter_32V_2A/HalfBridgeSw/GateDri2 ==
  Controlled Voltage Source : fl_lib/Electrical/Electrical Sources/Controlled Voltage Source
  Simulink-PS Converter : nesl_utility/Simulink-PS Converter  PhysicalDomain=network_engine_domain  SubClassName=ps_input  LeftPortType=input  RightPortType=output  PseudoPeriodic=off  Frequencies=[]  NoiseDistribution=none  NoiseParameters=[]  Unit=1  AffineConversion=off  FilteringAndDerivatives=provide  SimscapeFilterOrder=1  InputFilterTimeConstant=0.001  UdotUserProvided=0
  + : PMIOPort  Side=Left
  - : PMIOPort  Port=2  Side=Right
  wires:
  [bH] -> Simulink-PS Converter/1
  connections:
  Controlled Voltage Source/LConn1 -- +/RConn1
  Simulink-PS Converter/RConn1 -- Controlled Voltage Source/RConn1
  Controlled Voltage Source/RConn2 -- -/RConn1

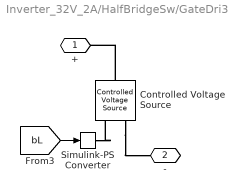
== system Inverter_32V_2A/HalfBridgeSw/GateDri3 ==
  Controlled Voltage Source : fl_lib/Electrical/Electrical Sources/Controlled Voltage Source
  Simulink-PS Converter : nesl_utility/Simulink-PS Converter  PhysicalDomain=network_engine_domain  SubClassName=ps_input  LeftPortType=input  RightPortType=output  PseudoPeriodic=off  Frequencies=[]  NoiseDistribution=none  NoiseParameters=[]  Unit=1  AffineConversion=off  FilteringAndDerivatives=provide  SimscapeFilterOrder=1  InputFilterTimeConstant=0.001  UdotUserProvided=0
  + : PMIOPort  Side=Left
  - : PMIOPort  Port=2  Side=Right
  wires:
  [bL] -> Simulink-PS Converter/1
  connections:
  Controlled Voltage Source/RConn2 -- -/RConn1
  Simulink-PS Converter/RConn1 -- Controlled Voltage Source/RConn1
  Controlled Voltage Source/LConn1 -- +/RConn1

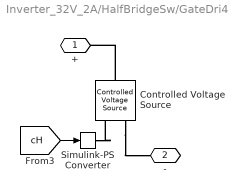
== system Inverter_32V_2A/HalfBridgeSw/GateDri4 ==
  Controlled Voltage Source : fl_lib/Electrical/Electrical Sources/Controlled Voltage Source
  Simulink-PS Converter : nesl_utility/Simulink-PS Converter  PhysicalDomain=network_engine_domain  SubClassName=ps_input  LeftPortType=input  RightPortType=output  PseudoPeriodic=off  Frequencies=[]  NoiseDistribution=none  NoiseParameters=[]  Unit=1  AffineConversion=off  FilteringAndDerivatives=provide  SimscapeFilterOrder=1  InputFilterTimeConstant=0.001  UdotUserProvided=0
  + : PMIOPort  Side=Left
  - : PMIOPort  Port=2  Side=Right
  wires:
  [cH] -> Simulink-PS Converter/1
  connections:
  Controlled Voltage Source/RConn2 -- -/RConn1
  Simulink-PS Converter/RConn1 -- Controlled Voltage Source/RConn1
  Controlled Voltage Source/LConn1 -- +/RConn1

== system Inverter_32V_2A/HalfBridgeSw/GateDri5 ==
  Controlled Voltage Source : fl_lib/Electrical/Electrical Sources/Controlled Voltage Source
  Simulink-PS Converter : nesl_utility/Simulink-PS Converter  PhysicalDomain=network_engine_domain  SubClassName=ps_input  LeftPortType=input  RightPortType=output  PseudoPeriodic=off  Frequencies=[]  NoiseDistribution=none  NoiseParameters=[]  Unit=1  AffineConversion=off  FilteringAndDerivatives=provide  SimscapeFilterOrder=1  InputFilterTimeConstant=0.001  UdotUserProvided=0
  + : PMIOPort  Side=Left
  - : PMIOPort  Port=2  Side=Right
  wires:
  [cL] -> Simulink-PS Converter/1
  connections:
  Controlled Voltage Source/LConn1 -- +/RConn1
  Simulink-PS Converter/RConn1 -- Controlled Voltage Source/RConn1
  Controlled Voltage Source/RConn2 -- -/RConn1
